simulink model "PassVeh14DOF"  (R2026b)
settings: Solver=ode23tb  StopTime=inf  FixedStep=.001  RelTol=1e-1  EnableMultiTasking=on
model workspace (MAT data in the model file):
  AlgnTrqCambCompl = [0 0 0 0]
  AlgnTrqSteerCompl = [0 0 0 0]
  AxlIxx = 62.3745166667
  AxlM = 160
  BumpCamber = [0 0 0 0]
  BumpCaster = [0 0 0 0]
  BumpSteer = [0 0 0 0]
  CambVsSteerAng = [0 0 0 0]
  CastVsSteerAng = [0 0 0 0]
  Cps = 2
  Cz = 5565.2246438
  CzWhlAxl = 11490.971257
  DCT_Param : object (value not decoded)
  Downshift_Speeds = [9.5625 12.9375 16.3125 19.6875 23.0625 26.4375 29.8125 33.1875 36.5625 39.9375 43.3125 46.6875 ... (28 elements, 4x7)]
  F0z = [2886 2907]
  F0zWhlAxl = 2907
  Hmax = 0.25
  Kz = 52451.0065793
  KzWhlAxl = 138031.612078
  LatCambCompl = [0 0 0 0]
  LatSteerCompl = [0 0 0 0]
  LatWhlCtrComplLat = [0 0 0 0]
  LatWhlCtrComplLng = [0  0  0  0; 0  0  0  0]
  LatWhlCtrDisp = [0 0 0 0]
  LngCambCompl = [0  0  0  0; 0  0  0  0]
  LngCastCompl = [0  0  0  0; 0  0  0  0]
  LngSteerCompl = [0  0  0  0; 0  0  0  0]
  LngWhlCtrCompl = [0  0  0  0; 0  0  0  0]
  LngWhlCtrDisp = [0 0 0 0]
  MotRatios = [1 1]
  NCyl = 6
  NrmlWhlFrcOff = [2886 2886 2907 2907]
  NrmlWhlRates = [52.4510065793 52.4510065793 52.4510065793 52.4510065793]
  Pedal_Positions = [0.1 0.4 0.5 0.9]
  Pstd = 101325
  Rair = 287
  RollCamber : object (value not decoded)
  RollCaster : object (value not decoded)
  RollSteer : object (value not decoded)
  RollStiffArb = [0 0]
  RollStiffArbFrnt = 800
  RollStiffNoArb = [0 0]
  RollStiffNoArbFrnt = 0
  RollStiffNoTwstRear = 0
  ShckFrcVsCompRate = [5.5652246438 5.5652246438 5.5652246438 5.5652246438]
  StatCamber = [0 0 0 0]
  StatCaster = [0 0 0 0]
  StatLdWhlR = [0.3 0.3 0.3 0.3]
  StatToe = [0 0 0 0]
  Trans : object (value not decoded)
  Tstd = 293.15
  Upshift_Speeds = [12.9375 16.3125 19.6875 33 26.4375 29.8125 33.1875 52.5 39.9375 43.3125 46.6875 77.25 ... (28 elements, 4x7)]
  VEH : object (value not decoded)
  Vd = 0.00346
  VrtLdTrnsfr = [0 0 0 0]
  WH : Mass (value not decoded)
  dt3D = 0.05
  f_air = [0 0 0 0 0 0 0 0 0 0 0 0 ... (256 elements, 16x16)]
  f_co = [0 0 0 0 0 0 0 0 0 0 0 0 ... (256 elements, 16x16)]
  f_co2 = [0 0 0 0 0 0 0 0 0 0 0 0 ... (256 elements, 16x16)]
  f_eff = [352.135682859 352.135682859 320.724378192 303.655312657 295.930136708 291.240087194 291.240271258 291.240312459 291.240275452 291.240198499 291.240100781 291.240018769 ... (256 elements, 16x16)]
  f_fuel = [0 0 0 0 0 0 0 0 0 0 0 0 ... (256 elements, 16x16)]
  f_hc = [0 0 0 0 0 0 0 0 0 0 0 0 ... (256 elements, 16x16)]
  f_nox = [0 0 0 0 0 0 0 0 0 0 0 0 ... (256 elements, 16x16)]
  f_pm = [0 0 0 0 0 0 0 0 0 0 0 0 ... (256 elements, 16x16)]
  f_susp_axl_bp = [1 2]
  f_susp_dz_bp = [-0.325022776267 -0.315022776267 -0.305022776267 -0.205022776267 -0.105022776267 -0.00502277626717 0.0949772237328 0.194977223733 0.204977223733 0.214977223733]
  f_susp_dzdot_bp = [-3 -0.3 -0.2 -0.1 0 0.1 0.2 0.3 3]
  f_susp_fmz = [-144070.391448 -93629.24037 -75929.1118915 -20630.5828179 -15385.48216 -10140.3815021 -4895.28084414 349.819813785 -31916.3973792 18437.6709544 -83996.1993354 -33555.0482577 ... (43920 elements, 10x9x61x2x4)]
  f_susp_geom = [0 0 0 0 0 0 0 0 0 0 0 0 ... (3660 elements, 10x61x2x3)]
  f_susp_strgdelta_bp = [-0.523598775598 -0.506145483078 -0.488692190558 -0.471238898038 -0.453785605519 -0.436332312999 -0.418879020479 -0.401425727959 -0.383972435439 -0.366519142919 -0.349065850399 -0.331612557879 ... (61 elements, 1x61)]
  f_tbrake = [0 76.8593923996 105.140482948 131.533638111 157.926793274 176.658631717 176.65727296 176.656856686 176.656879077 176.657093756 176.657404516 176.65772406 ... (256 elements, 16x16)]
  f_tbrake_n_bpt = [0 649.519052838 912.419621844 1175.32019085 1438.22075986 1701.12132886 1964.02189787 2226.92246687 2489.82303588 2752.72360489 3015.62417389 3278.5247429 ... (16 elements, 1x16)]
  f_tbrake_t_bpt = [0 34.6410161514 61.0341713143 87.4273264773 113.82048164 140.213636803 166.606791966 192.999947129 219.393102292 245.786257455 272.179412618 298.572567781 ... (16 elements, 1x16)]
  f_texh = [766.752464599 766.752464599 786.17542386 801.679939032 884.591982581 910.574397722 910.571871054 910.570774534 910.570601632 910.570821151 910.571247242 910.571639815 ... (256 elements, 16x16)]
  f_twc_eff_co = [0.17 0.25 0.45 0.99 0.99 0.99 0.99]
  f_twc_eff_hc = [0.21 0.375 0.75 0.98 0.98 0.98 0.98]
  f_twc_eff_lam = [0.909090909 0.944055944 0.979020979 1 1.013986014 1.048951049 1.083916084]
  f_twc_eff_nox = [0.98 0.98 0.98 0.97 0.05 0.02 0]
  numWheel = 4
symbols that are objects in the model workspace (value not decoded): VEH
libraries: vehdynlibtire x12, vehdynlibsuspension x8, autolibutils x5, sharedtransform x5, shared6dof x2, vehdynlibeom x1, vehdynlibtirecommon x1, matrix_library x1
(part 3 of 9)

== system PassVeh14DOF/Wheels and Tires/VDBS ==
  WhlAng : Inport
  WhlCmb : Inport  Port=2  Unit=rad
  AxleTrq : Inport  Port=3
  BrkPrs : Inport  Port=4
  Fz : Inport  Port=5  Unit=N
  r : Inport  Port=6
  VehVel : Inport  Port=7
  Ground Level : Inport  Port=8
  DCM : Inport  Port=9
  Friction : Inport  Port=10  Unit=1  PortDimensions=4
  Veh : Inport  Port=11
  Pressure : vehdynlibtirecommon/Constant  const=220000  numWheels=4
  Scale Factors : vehdynlibtire/Scale Factors  numWhls=4  LFZO=1  input_LFZO=off  LMUX=1  input_LMUX=on  LMUY=1  input_LMUY=on  LMUV=0  input_LMUV=off  LKX=1  input_LKX=off  LKY=1  input_LKY=off  LCX=1  input_LCX=off  LCY=1  input_LCY=off  LEX=1  input_LEX=off  LEY=1  input_LEY=off  LHX=1  input_LHX=off  LHY=1  input_LHY=off  LVX=1  input_LVX=off  LVY=1  input_LVY=off  LKYC=1  input_LKYC=off  LKZC=1  input_LKZC=off  LTR=1  input_LTR=off  LRES=1  input_LRES=off  LXAL=1  input_LXAL=off  LYKA=1  input_LYKA=off  LVYKA=1  input_LVYKA=off  LS=1  input_LS=off  LCZ=1  input_LCZ=off  LMX=1  input_LMX=off  LVMX=1  input_LVMX=off  LMY=1  input_LMY=off  LMP=1  input_LMP=off
  Terminator : Terminator
  Tire2Veh : Subsystem
  Tires : Subsystem  Variant=on  VariantControlMode=label  VariantControl=Variant1  LabelModeActiveChoice=2
  Veh2Tire : Subsystem
  Wheels : Outport  VectorParamsAs1DForOutWhenUnconnected=off
  Wheels2Susp : Outport  Port=2  VectorParamsAs1DForOutWhenUnconnected=off
  FrntAxlF : Outport  Port=3  Unit=N  VectorParamsAs1DForOutWhenUnconnected=off
  RearAxlF : Outport  Port=4  Unit=N  VectorParamsAs1DForOutWhenUnconnected=off
  Omega : Outport  Port=5  VectorParamsAs1DForOutWhenUnconnected=off
  Mz : Outport  Port=6  Unit=N*m  VectorParamsAs1DForOutWhenUnconnected=off
  SuspWhlPz : Outport  Port=7  VectorParamsAs1DForOutWhenUnconnected=off
  SuspWhlVz : Outport  Port=8  VectorParamsAs1DForOutWhenUnconnected=off
  wires:
  Ground Level/1 -> Tires/9("Gnd ")
  Pressure/1 -> Tires/7("Press ")
  Scale Factors/1 -> Tires/8("lambda ")
  Fz/1 -> Tire2Veh/3(Fz), Tires/10("FzSusp ")
  AxleTrq/1 -> Veh2Tire/2(Axle)
  BrkPrs/1 -> Veh2Tire/3(Brake)
  VehVel/1 -> Veh2Tire/4(VehVel)
  Veh2Tire/1(T) -> Tires/1("DriveTorque ")
  Veh2Tire/2(P) -> Tires/2("Brake Pressure ")
  Veh2Tire/4(xdotAxle) -> Tires/4("Vx ")
  Veh2Tire/5(ydotAxle) -> Tires/5("Vy ")
  Veh2Tire/3(psidot) -> Tires/3("r ")
  WhlAng/1 -> Tire2Veh/6(WhlAng), Veh2Tire/5(WhlAng)
  Tire2Veh/3(Omega) -> Omega/1
  Tire2Veh/4(FrntAxlF) -> FrntAxlF/1
  Tire2Veh/5(RearAxlF) -> RearAxlF/1
  Tire2Veh/6(<Mz>) -> Mz/1
  Friction/1 -> Scale Factors/2, Scale Factors/1
  r/1 -> Veh2Tire/1(r)
  Veh2Tire/6(zdotAxle) -> Terminator/1
  Tire2Veh/7(SuspWhlPz) -> SuspWhlPz/1
  Tire2Veh/8(SuspWhlVz) -> SuspWhlVz/1
  Veh/1 -> Tire2Veh/1(Veh)
  Tire2Veh/2(Wheels2Susp) -> Wheels2Susp/1
  Tires/1(" Wheels") -> Tire2Veh/2(Wheels)  "TireFrame"
  Tire2Veh/1(Wheel) -> Wheels/1
  WhlCmb/1 -> Veh2Tire/6(WhlCmb), Tire2Veh/5(WhlCmb)  "WhlCamberIn"
  Veh2Tire/7(Camber) -> Tires/6("Camber ")
  DCM/1 -> Veh2Tire/7(DCM), Tire2Veh/4(DCM)

== system PassVeh14DOF/Suspension/Double Wishbone Suspension/Steer Rate Adapter ==
  Veh : Inport
  Add : Sum
  Bus Selector3 : BusSelector  OutputSignals=BdyFrm.Cg.AngVel.r
  Constant : Constant  Value=zeros(1,4)
  Matrix Concatenate : Concatenate  NumInputs=3  Mode=Multidimensional array
  Matrix Concatenate1 : Concatenate  NumInputs=3  Mode=Multidimensional array
  Reshape2 : Reshape  OutputDimensionality=Row vector (2-D)
  Reshape3 : Reshape  OutputDimensionality=Row vector (2-D)
  Reshape4 : Reshape  OutputDimensionality=Row vector (2-D)
  Selector3 : Selector  InputPortWidth=1  IndexOptions=Index vector (dialog)  Indices=[1 1 1 1]  OutputSizes=1
  SteerRates : Constant  Value=zeros(1,4)
  AngVel : Outport  VectorParamsAs1DForOutWhenUnconnected=off
  wires:
  Reshape2/1 -> Matrix Concatenate1/1, Matrix Concatenate1/3, Matrix Concatenate1/2
  Constant/1 -> Reshape3/1
  Selector3/1 -> Reshape4/1
  Bus Selector3/1 -> Selector3/1  "<r>"
  Matrix Concatenate/1 -> Add/2
  SteerRates/1 -> Reshape2/1
  Reshape4/1 -> Matrix Concatenate/3
  Reshape3/1 -> Matrix Concatenate/2, Matrix Concatenate/1
  Matrix Concatenate1/1 -> Add/1
  Veh/1 -> Bus Selector3/1
  Add/1 -> AngVel/1  "AngVel"

== system PassVeh14DOF/Suspension/Double Wishbone Suspension/Steering Adapter ==
  Steer : Inport
  Reshape1 : Reshape  OutputDimensionality=Row vector (2-D)
  Selector : Selector  IndexOptions=Index vector (dialog)  Indices=[1 2]  OutputSizes=1
  StrgAng : Outport  VectorParamsAs1DForOutWhenUnconnected=off
  wires:
  Reshape1/1 -> StrgAng/1
  Steer/1 -> Selector/1
  Selector/1 -> Reshape1/1

== system PassVeh14DOF/Suspension/Double Wishbone Suspension/Vehicle Adapter ==
  Veh : Inport
  Bus Creator3 : BusCreator  Inputs=2
  Bus Selector1 : BusSelector  OutputSignals=InertFrm.FrntAxl.Lft.Disp.X,InertFrm.FrntAxl.Lft.Disp.Y,InertFrm.FrntAxl.Lft.Disp.Z,InertFrm.FrntAxl.Rght.Disp.X,InertFrm.FrntAxl.Rght.Disp.Y,InertFrm.FrntAxl.Rght.Disp.Z,InertFrm.RearAxl.Lft.Disp.X,InertFrm.RearAxl.Lft.Disp.Y,InertFrm.RearAxl.Lft.Disp.Z,InertFrm.RearAxl.Rght.Disp.X,InertFrm.RearAxl.Rght.Disp.Y,InertFrm.RearAxl.Rght.Disp.Z
  Bus Selector2 : BusSelector  OutputSignals=BdyFrm.FrntAxl.Lft.Vel.xdot,BdyFrm.FrntAxl.Lft.Vel.ydot,BdyFrm.FrntAxl.Lft.Vel.zdot,BdyFrm.FrntAxl.Rght.Vel.xdot,BdyFrm.FrntAxl.Rght.Vel.ydot,BdyFrm.FrntAxl.Rght.Vel.zdot,BdyFrm.RearAxl.Lft.Vel.xdot,BdyFrm.RearAxl.Lft.Vel.ydot,BdyFrm.RearAxl.Lft.Vel.zdot,BdyFrm.RearAxl.Rght.Vel.xdot,BdyFrm.RearAxl.Rght.Vel.ydot,BdyFrm.RearAxl.Rght.Vel.zdot
  Bus Selector3 : BusSelector  OutputSignals=InertFrm.FrntAxl.Lft.Vel.Xdot,InertFrm.FrntAxl.Lft.Vel.Ydot,InertFrm.FrntAxl.Lft.Vel.Zdot,InertFrm.FrntAxl.Rght.Vel.Xdot,InertFrm.FrntAxl.Rght.Vel.Ydot,InertFrm.FrntAxl.Rght.Vel.Zdot,InertFrm.RearAxl.Lft.Vel.Xdot,InertFrm.RearAxl.Lft.Vel.Ydot,InertFrm.RearAxl.Lft.Vel.Zdot,InertFrm.RearAxl.Rght.Vel.Xdot,InertFrm.RearAxl.Rght.Vel.Ydot,InertFrm.RearAxl.Rght.Vel.Zdot
  Inertial Frame CG to Axle Offset : Constant  Value=[zeros(2,4);VEH.HeightCG*ones(1,4)]
  Mux1 : Mux  Inputs=12
  Mux2 : Mux  Inputs=12
  Mux3 : Mux  Inputs=12
  Reshape : Reshape  OutputDimensionality=Customize  OutputDimensions=[3,4]
  Reshape1 : Reshape  OutputDimensionality=Customize  OutputDimensions=[3,4]
  Reshape2 : Reshape  OutputDimensionality=Customize  OutputDimensions=[3,4]
  Sum : Sum  Inputs=|+-
  VehSusp : Outport  VectorParamsAs1DForOutWhenUnconnected=off
  VehVbody : Outport  Port=2  VectorParamsAs1DForOutWhenUnconnected=off
  wires:
  Veh/1 -> Bus Selector3/1, Bus Selector2/1, Bus Selector1/1
  Reshape2/1 -> VehVbody/1  "V"
  Bus Creator3/1 -> VehSusp/1  "Veh"
  Reshape/1 -> Sum/1
  Bus Selector1/1 -> Mux2/1  "<X>"
  Bus Selector1/2 -> Mux2/2  "<Y>"
  Bus Selector1/3 -> Mux2/3  "<Z>"
  Bus Selector1/4 -> Mux2/4  "<X>"
  Bus Selector1/5 -> Mux2/5  "<Y>"
  Bus Selector1/6 -> Mux2/6  "<Z>"
  Bus Selector1/7 -> Mux2/7  "<X>"
  Bus Selector1/8 -> Mux2/8  "<Y>"
  Bus Selector1/9 -> Mux2/9  "<Z>"
  Bus Selector1/10 -> Mux2/10  "<X>"
  Bus Selector1/11 -> Mux2/11  "<Y>"
  Bus Selector1/12 -> Mux2/12  "<Z>"
  Bus Selector2/1 -> Mux1/1  "<xdot>"
  Bus Selector2/2 -> Mux1/2  "<ydot>"
  Bus Selector2/3 -> Mux1/3  "<zdot>"
  Bus Selector2/4 -> Mux1/4  "<xdot>"
  Bus Selector2/5 -> Mux1/5  "<ydot>"
  Bus Selector2/6 -> Mux1/6  "<zdot>"
  Bus Selector2/7 -> Mux1/7  "<xdot>"
  Bus Selector2/8 -> Mux1/8  "<ydot>"
  Bus Selector2/9 -> Mux1/9  "<zdot>"
  Bus Selector2/10 -> Mux1/10  "<xdot>"
  Bus Selector2/11 -> Mux1/11  "<ydot>"
  Bus Selector2/12 -> Mux1/12  "<zdot>"
  Mux1/1 -> Reshape2/1
  Mux2/1 -> Reshape/1
  Inertial Frame CG to Axle Offset/1 -> Sum/2
  Sum/1 -> Bus Creator3/1  "P"
  Mux3/1 -> Reshape1/1
  Bus Selector3/12 -> Mux3/12  "<Zdot>"
  Bus Selector3/11 -> Mux3/11  "<Ydot>"
  Bus Selector3/10 -> Mux3/10  "<Xdot>"
  Bus Selector3/9 -> Mux3/9  "<Zdot>"
  Bus Selector3/8 -> Mux3/8  "<Ydot>"
  Bus Selector3/7 -> Mux3/7  "<Xdot>"
  Bus Selector3/6 -> Mux3/6  "<Zdot>"
  Bus Selector3/5 -> Mux3/5  "<Ydot>"
  Bus Selector3/4 -> Mux3/4  "<Xdot>"
  Bus Selector3/3 -> Mux3/3  "<Zdot>"
  Bus Selector3/2 -> Mux3/2  "<Ydot>"
  Bus Selector3/1 -> Mux3/1  "<Xdot>"
  Reshape1/1 -> Bus Creator3/2  "V"

== system PassVeh14DOF/Suspension/Double Wishbone Suspension/Wheel  Adapter ==
  Wheels : Inport
  Bus Selector : BusSelector  OutputSignals=SuspFrame.Fx,SuspFrame.Fy
  Bus Selector1 : BusSelector  OutputSignals=SuspFrame.RL
  Bus Selector2 : BusSelector  OutputSignals=SuspFrame.Mx,SuspFrame.My,SuspFrame.Mz
  Bus Selector3 : BusSelector  OutputSignals=SuspFrame.z,SuspFrame.zdot
  Matrix Concatenate : Concatenate  NumInputs=3  Mode=Multidimensional array
  Reshape{,1..7} (8 alike) : Reshape  OutputDimensionality=Row vector (2-D)
  WhlFx : Outport  VectorParamsAs1DForOutWhenUnconnected=off
  WhlFy : Outport  Port=2  VectorParamsAs1DForOutWhenUnconnected=off
  z : Outport  Port=3  VectorParamsAs1DForOutWhenUnconnected=off
  zdot : Outport  Port=4  VectorParamsAs1DForOutWhenUnconnected=off
  M : Outport  Port=5  VectorParamsAs1DForOutWhenUnconnected=off
  RL : Outport  Port=6  VectorParamsAs1DForOutWhenUnconnected=off
  wires:
  Reshape7/1 -> WhlFy/1
  Reshape6/1 -> WhlFx/1
  Bus Selector/1 -> Reshape6/1  "<Fx>"
  Bus Selector/2 -> Reshape7/1  "<Fy>"
  Bus Selector3/1 -> Reshape/1  "<z>"
  Wheels/1 -> Bus Selector1/1, Bus Selector2/1, Bus Selector3/1, Bus Selector/1
  Bus Selector3/2 -> Reshape2/1  "<zdot>"
  Reshape2/1 -> zdot/1  "zdot"
  Bus Selector1/1 -> Reshape1/1  "<RL>"
  Reshape1/1 -> RL/1  "RL"
  Bus Selector2/1 -> Reshape3/1  "<Mx>"
  Bus Selector2/2 -> Reshape4/1  "<My>"
  Bus Selector2/3 -> Reshape5/1  "<Mz>"
  Reshape3/1 -> Matrix Concatenate/1
  Reshape4/1 -> Matrix Concatenate/2
  Reshape5/1 -> Matrix Concatenate/3
  Matrix Concatenate/1 -> M/1  "M"
  Reshape/1 -> z/1  "z"

== system PassVeh14DOF/Suspension/Independent Mapped Front Suspension Mapped Solid Axle Rear Suspension/Steer Rate Adapter ==
  Veh : Inport
  Add : Sum
  Bus Selector3 : BusSelector  OutputSignals=BdyFrm.Cg.AngVel.r
  Constant : Constant  Value=zeros(1,4)
  Matrix Concatenate : Concatenate  NumInputs=3  Mode=Multidimensional array
  Matrix Concatenate1 : Concatenate  NumInputs=3  Mode=Multidimensional array
  Reshape2 : Reshape  OutputDimensionality=Row vector (2-D)
  Reshape3 : Reshape  OutputDimensionality=Row vector (2-D)
  Reshape4 : Reshape  OutputDimensionality=Row vector (2-D)
  Selector3 : Selector  InputPortWidth=1  IndexOptions=Index vector (dialog)  Indices=[1 1 1 1]  OutputSizes=1
  SteerRates : Constant  Value=zeros(1,4)
  AngVel : Outport  VectorParamsAs1DForOutWhenUnconnected=off
  wires:
  Reshape2/1 -> Matrix Concatenate1/1, Matrix Concatenate1/3, Matrix Concatenate1/2
  Constant/1 -> Reshape3/1
  Selector3/1 -> Reshape4/1
  Bus Selector3/1 -> Selector3/1  "<r>"
  Matrix Concatenate/1 -> Add/2
  SteerRates/1 -> Reshape2/1
  Reshape4/1 -> Matrix Concatenate/3
  Reshape3/1 -> Matrix Concatenate/2, Matrix Concatenate/1
  Matrix Concatenate1/1 -> Add/1
  Veh/1 -> Bus Selector3/1
  Add/1 -> AngVel/1  "AngVel"

== system PassVeh14DOF/Suspension/Independent Mapped Front Suspension Mapped Solid Axle Rear Suspension/Steering Adapter ==
  Steer : Inport
  Reshape1 : Reshape  OutputDimensionality=Row vector (2-D)
  Selector : Selector  IndexOptions=Index vector (dialog)  Indices=[1 2]  OutputSizes=1
  StrgAng : Outport  VectorParamsAs1DForOutWhenUnconnected=off
  wires:
  Reshape1/1 -> StrgAng/1
  Steer/1 -> Selector/1
  Selector/1 -> Reshape1/1

== system PassVeh14DOF/Suspension/Independent Mapped Front Suspension Mapped Solid Axle Rear Suspension/Vehicle Adapter ==
  Veh : Inport
  Bus Creator3 : BusCreator  Inputs=2
  Bus Selector1 : BusSelector  OutputSignals=InertFrm.FrntAxl.Lft.Disp.X,InertFrm.FrntAxl.Lft.Disp.Y,InertFrm.FrntAxl.Lft.Disp.Z,InertFrm.FrntAxl.Rght.Disp.X,InertFrm.FrntAxl.Rght.Disp.Y,InertFrm.FrntAxl.Rght.Disp.Z,InertFrm.RearAxl.Lft.Disp.X,InertFrm.RearAxl.Lft.Disp.Y,InertFrm.RearAxl.Lft.Disp.Z,InertFrm.RearAxl.Rght.Disp.X,InertFrm.RearAxl.Rght.Disp.Y,InertFrm.RearAxl.Rght.Disp.Z
  Bus Selector2 : BusSelector  OutputSignals=BdyFrm.FrntAxl.Lft.Vel.xdot,BdyFrm.FrntAxl.Lft.Vel.ydot,BdyFrm.FrntAxl.Lft.Vel.zdot,BdyFrm.FrntAxl.Rght.Vel.xdot,BdyFrm.FrntAxl.Rght.Vel.ydot,BdyFrm.FrntAxl.Rght.Vel.zdot,BdyFrm.RearAxl.Lft.Vel.xdot,BdyFrm.RearAxl.Lft.Vel.ydot,BdyFrm.RearAxl.Lft.Vel.zdot,BdyFrm.RearAxl.Rght.Vel.xdot,BdyFrm.RearAxl.Rght.Vel.ydot,BdyFrm.RearAxl.Rght.Vel.zdot
  Bus Selector3 : BusSelector  OutputSignals=InertFrm.FrntAxl.Lft.Vel.Xdot,InertFrm.FrntAxl.Lft.Vel.Ydot,InertFrm.FrntAxl.Lft.Vel.Zdot,InertFrm.FrntAxl.Rght.Vel.Xdot,InertFrm.FrntAxl.Rght.Vel.Ydot,InertFrm.FrntAxl.Rght.Vel.Zdot,InertFrm.RearAxl.Lft.Vel.Xdot,InertFrm.RearAxl.Lft.Vel.Ydot,InertFrm.RearAxl.Lft.Vel.Zdot,InertFrm.RearAxl.Rght.Vel.Xdot,InertFrm.RearAxl.Rght.Vel.Ydot,InertFrm.RearAxl.Rght.Vel.Zdot
  Inertial Frame CG to Axle Offset : Constant  Value=[zeros(2,4);VEH.HeightCG*ones(1,4)]
  Mux1 : Mux  Inputs=12
  Mux2 : Mux  Inputs=12
  Mux3 : Mux  Inputs=12
  Reshape : Reshape  OutputDimensionality=Customize  OutputDimensions=[3,4]
  Reshape1 : Reshape  OutputDimensionality=Customize  OutputDimensions=[3,4]
  Reshape2 : Reshape  OutputDimensionality=Customize  OutputDimensions=[3,4]
  Sum : Sum  Inputs=|+-
  VehSusp : Outport  VectorParamsAs1DForOutWhenUnconnected=off
  VehVbody : Outport  Port=2  VectorParamsAs1DForOutWhenUnconnected=off
  wires:
  Veh/1 -> Bus Selector3/1, Bus Selector2/1, Bus Selector1/1
  Reshape2/1 -> VehVbody/1  "V"
  Bus Creator3/1 -> VehSusp/1  "Veh"
  Reshape/1 -> Sum/1
  Bus Selector1/1 -> Mux2/1  "<X>"
  Bus Selector1/2 -> Mux2/2  "<Y>"
  Bus Selector1/3 -> Mux2/3  "<Z>"
  Bus Selector1/4 -> Mux2/4  "<X>"
  Bus Selector1/5 -> Mux2/5  "<Y>"
  Bus Selector1/6 -> Mux2/6  "<Z>"
  Bus Selector1/7 -> Mux2/7  "<X>"
  Bus Selector1/8 -> Mux2/8  "<Y>"
  Bus Selector1/9 -> Mux2/9  "<Z>"
  Bus Selector1/10 -> Mux2/10  "<X>"
  Bus Selector1/11 -> Mux2/11  "<Y>"
  Bus Selector1/12 -> Mux2/12  "<Z>"
  Bus Selector2/1 -> Mux1/1  "<xdot>"
  Bus Selector2/2 -> Mux1/2  "<ydot>"
  Bus Selector2/3 -> Mux1/3  "<zdot>"
  Bus Selector2/4 -> Mux1/4  "<xdot>"
  Bus Selector2/5 -> Mux1/5  "<ydot>"
  Bus Selector2/6 -> Mux1/6  "<zdot>"
  Bus Selector2/7 -> Mux1/7  "<xdot>"
  Bus Selector2/8 -> Mux1/8  "<ydot>"
  Bus Selector2/9 -> Mux1/9  "<zdot>"
  Bus Selector2/10 -> Mux1/10  "<xdot>"
  Bus Selector2/11 -> Mux1/11  "<ydot>"
  Bus Selector2/12 -> Mux1/12  "<zdot>"
  Mux1/1 -> Reshape2/1
  Mux2/1 -> Reshape/1
  Inertial Frame CG to Axle Offset/1 -> Sum/2
  Sum/1 -> Bus Creator3/1  "P"
  Mux3/1 -> Reshape1/1
  Bus Selector3/12 -> Mux3/12  "<Zdot>"
  Bus Selector3/11 -> Mux3/11  "<Ydot>"
  Bus Selector3/10 -> Mux3/10  "<Xdot>"
  Bus Selector3/9 -> Mux3/9  "<Zdot>"
  Bus Selector3/8 -> Mux3/8  "<Ydot>"
  Bus Selector3/7 -> Mux3/7  "<Xdot>"
  Bus Selector3/6 -> Mux3/6  "<Zdot>"
  Bus Selector3/5 -> Mux3/5  "<Ydot>"
  Bus Selector3/4 -> Mux3/4  "<Xdot>"
  Bus Selector3/3 -> Mux3/3  "<Zdot>"
  Bus Selector3/2 -> Mux3/2  "<Ydot>"
  Bus Selector3/1 -> Mux3/1  "<Xdot>"
  Reshape1/1 -> Bus Creator3/2  "V"

== system PassVeh14DOF/Suspension/Independent Mapped Front Suspension Mapped Solid Axle Rear Suspension/Wheel  Adapter ==
  Wheels : Inport
  Bus Selector : BusSelector  OutputSignals=SuspFrame.Fx,SuspFrame.Fy
  Bus Selector1 : BusSelector  OutputSignals=SuspFrame.RL
  Bus Selector2 : BusSelector  OutputSignals=SuspFrame.Mx,SuspFrame.My,SuspFrame.Mz
  Bus Selector3 : BusSelector  OutputSignals=SuspFrame.z,SuspFrame.zdot
  Matrix Concatenate : Concatenate  NumInputs=3  Mode=Multidimensional array
  Reshape{,1..7} (8 alike) : Reshape  OutputDimensionality=Row vector (2-D)
  WhlFx : Outport  VectorParamsAs1DForOutWhenUnconnected=off
  WhlFy : Outport  Port=2  VectorParamsAs1DForOutWhenUnconnected=off
  z : Outport  Port=3  VectorParamsAs1DForOutWhenUnconnected=off
  zdot : Outport  Port=4  VectorParamsAs1DForOutWhenUnconnected=off
  M : Outport  Port=5  VectorParamsAs1DForOutWhenUnconnected=off
  RL : Outport  Port=6  VectorParamsAs1DForOutWhenUnconnected=off
  wires:
  Reshape7/1 -> WhlFy/1
  Reshape6/1 -> WhlFx/1
  Bus Selector/1 -> Reshape6/1  "<Fx>"
  Bus Selector/2 -> Reshape7/1  "<Fy>"
  Bus Selector3/1 -> Reshape/1  "<z>"
  Wheels/1 -> Bus Selector1/1, Bus Selector2/1, Bus Selector3/1, Bus Selector/1
  Bus Selector3/2 -> Reshape2/1  "<zdot>"
  Reshape2/1 -> zdot/1  "zdot"
  Bus Selector1/1 -> Reshape1/1  "<RL>"
  Reshape1/1 -> RL/1  "RL"
  Bus Selector2/1 -> Reshape3/1  "<Mx>"
  Bus Selector2/2 -> Reshape4/1  "<My>"
  Bus Selector2/3 -> Reshape5/1  "<Mz>"
  Reshape3/1 -> Matrix Concatenate/1
  Reshape4/1 -> Matrix Concatenate/2
  Reshape5/1 -> Matrix Concatenate/3
  Matrix Concatenate/1 -> M/1  "M"
  Reshape/1 -> z/1  "z"

== system PassVeh14DOF/Suspension/Kinematics and Compliance Independent Suspension/Calculate dynamic track width from lateral wheel center displacement change ==
  dWhlY : Inport
  dWhlZ : Inport  Port=2
  Front Track Calculation : Subsystem
  Gain : Gain  Gain=-1
  Rear Track Calculation : Subsystem
  Sign : Signum  ZeroCross=off
  Vector Concatenate : Concatenate
  w : Outport
  wires:
  dWhlZ/1 -> Gain/1
  dWhlY/1 -> Rear Track Calculation/1(dWhlY), Front Track Calculation/1(dWhlY)
  Vector Concatenate/1 -> w/1
  Front Track Calculation/1(w_front) -> Vector Concatenate/1
  Rear Track Calculation/1(w_rear) -> Vector Concatenate/2
  Sign/1 -> Rear Track Calculation/2(sign), Front Track Calculation/2(sign)
  Gain/1 -> Sign/1

== system PassVeh14DOF/Suspension/Kinematics and Compliance Independent Suspension/Steer Rate Adapter ==
  Veh : Inport
  Add : Sum
  Bus Selector3 : BusSelector  OutputSignals=BdyFrm.Cg.AngVel.r
  Constant : Constant  Value=zeros(1,4)
  Matrix Concatenate : Concatenate  NumInputs=3  Mode=Multidimensional array
  Matrix Concatenate1 : Concatenate  NumInputs=3  Mode=Multidimensional array
  Reshape2 : Reshape  OutputDimensionality=Row vector (2-D)
  Reshape3 : Reshape  OutputDimensionality=Row vector (2-D)
  Reshape4 : Reshape  OutputDimensionality=Row vector (2-D)
  Selector3 : Selector  InputPortWidth=1  IndexOptions=Index vector (dialog)  Indices=[1 1 1 1]  OutputSizes=1
  SteerRates : Constant  Value=zeros(1,4)
  AngVel : Outport  VectorParamsAs1DForOutWhenUnconnected=off
  wires:
  Reshape2/1 -> Matrix Concatenate1/1, Matrix Concatenate1/3, Matrix Concatenate1/2
  Constant/1 -> Reshape3/1
  Selector3/1 -> Reshape4/1
  Bus Selector3/1 -> Selector3/1  "<r>"
  Matrix Concatenate/1 -> Add/2
  SteerRates/1 -> Reshape2/1
  Reshape4/1 -> Matrix Concatenate/3
  Reshape3/1 -> Matrix Concatenate/2, Matrix Concatenate/1
  Matrix Concatenate1/1 -> Add/1
  Veh/1 -> Bus Selector3/1
  Add/1 -> AngVel/1  "AngVel"

== system PassVeh14DOF/Suspension/Kinematics and Compliance Independent Suspension/Steering Adapter ==
  Steer : Inport
  Reshape1 : Reshape  OutputDimensionality=Row vector (2-D)
  Selector : Selector  IndexOptions=Index vector (dialog)  Indices=[1 2]  OutputSizes=1
  StrgAng : Outport  VectorParamsAs1DForOutWhenUnconnected=off
  wires:
  Reshape1/1 -> StrgAng/1
  Steer/1 -> Selector/1
  Selector/1 -> Reshape1/1

== system PassVeh14DOF/Suspension/Kinematics and Compliance Independent Suspension/Vehicle Adapter ==
  Veh : Inport
  Bus Creator3 : BusCreator  Inputs=2
  Bus Selector1 : BusSelector  OutputSignals=InertFrm.FrntAxl.Lft.Disp.X,InertFrm.FrntAxl.Lft.Disp.Y,InertFrm.FrntAxl.Lft.Disp.Z,InertFrm.FrntAxl.Rght.Disp.X,InertFrm.FrntAxl.Rght.Disp.Y,InertFrm.FrntAxl.Rght.Disp.Z,InertFrm.RearAxl.Lft.Disp.X,InertFrm.RearAxl.Lft.Disp.Y,InertFrm.RearAxl.Lft.Disp.Z,InertFrm.RearAxl.Rght.Disp.X,InertFrm.RearAxl.Rght.Disp.Y,InertFrm.RearAxl.Rght.Disp.Z
  Bus Selector2 : BusSelector  OutputSignals=BdyFrm.FrntAxl.Lft.Vel.xdot,BdyFrm.FrntAxl.Lft.Vel.ydot,BdyFrm.FrntAxl.Lft.Vel.zdot,BdyFrm.FrntAxl.Rght.Vel.xdot,BdyFrm.FrntAxl.Rght.Vel.ydot,BdyFrm.FrntAxl.Rght.Vel.zdot,BdyFrm.RearAxl.Lft.Vel.xdot,BdyFrm.RearAxl.Lft.Vel.ydot,BdyFrm.RearAxl.Lft.Vel.zdot,BdyFrm.RearAxl.Rght.Vel.xdot,BdyFrm.RearAxl.Rght.Vel.ydot,BdyFrm.RearAxl.Rght.Vel.zdot
  Bus Selector3 : BusSelector  OutputSignals=InertFrm.FrntAxl.Lft.Vel.Xdot,InertFrm.FrntAxl.Lft.Vel.Ydot,InertFrm.FrntAxl.Lft.Vel.Zdot,InertFrm.FrntAxl.Rght.Vel.Xdot,InertFrm.FrntAxl.Rght.Vel.Ydot,InertFrm.FrntAxl.Rght.Vel.Zdot,InertFrm.RearAxl.Lft.Vel.Xdot,InertFrm.RearAxl.Lft.Vel.Ydot,InertFrm.RearAxl.Lft.Vel.Zdot,InertFrm.RearAxl.Rght.Vel.Xdot,InertFrm.RearAxl.Rght.Vel.Ydot,InertFrm.RearAxl.Rght.Vel.Zdot
  Inertial Frame CG to Axle Offset : Constant  Value=[zeros(2,4);VEH.HeightCG*ones(1,4)]
  Mux1 : Mux  Inputs=12
  Mux2 : Mux  Inputs=12
  Mux3 : Mux  Inputs=12
  Reshape : Reshape  OutputDimensionality=Customize  OutputDimensions=[3,4]
  Reshape1 : Reshape  OutputDimensionality=Customize  OutputDimensions=[3,4]
  Reshape2 : Reshape  OutputDimensionality=Customize  OutputDimensions=[3,4]
  Sum : Sum  Inputs=|+-
  VehSusp : Outport  VectorParamsAs1DForOutWhenUnconnected=off
  VehVbody : Outport  Port=2  VectorParamsAs1DForOutWhenUnconnected=off
  wires:
  Veh/1 -> Bus Selector3/1, Bus Selector2/1, Bus Selector1/1
  Reshape2/1 -> VehVbody/1  "V"
  Bus Creator3/1 -> VehSusp/1  "Veh"
  Reshape/1 -> Sum/1
  Bus Selector1/1 -> Mux2/1  "<X>"
  Bus Selector1/2 -> Mux2/2  "<Y>"
  Bus Selector1/3 -> Mux2/3  "<Z>"
  Bus Selector1/4 -> Mux2/4  "<X>"
  Bus Selector1/5 -> Mux2/5  "<Y>"
  Bus Selector1/6 -> Mux2/6  "<Z>"
  Bus Selector1/7 -> Mux2/7  "<X>"
  Bus Selector1/8 -> Mux2/8  "<Y>"
  Bus Selector1/9 -> Mux2/9  "<Z>"
  Bus Selector1/10 -> Mux2/10  "<X>"
  Bus Selector1/11 -> Mux2/11  "<Y>"
  Bus Selector1/12 -> Mux2/12  "<Z>"
  Bus Selector2/1 -> Mux1/1  "<xdot>"
  Bus Selector2/2 -> Mux1/2  "<ydot>"
  Bus Selector2/3 -> Mux1/3  "<zdot>"
  Bus Selector2/4 -> Mux1/4  "<xdot>"
  Bus Selector2/5 -> Mux1/5  "<ydot>"
  Bus Selector2/6 -> Mux1/6  "<zdot>"
  Bus Selector2/7 -> Mux1/7  "<xdot>"
  Bus Selector2/8 -> Mux1/8  "<ydot>"
  Bus Selector2/9 -> Mux1/9  "<zdot>"
  Bus Selector2/10 -> Mux1/10  "<xdot>"
  Bus Selector2/11 -> Mux1/11  "<ydot>"
  Bus Selector2/12 -> Mux1/12  "<zdot>"
  Mux1/1 -> Reshape2/1
  Mux2/1 -> Reshape/1
  Inertial Frame CG to Axle Offset/1 -> Sum/2
  Sum/1 -> Bus Creator3/1  "P"
  Mux3/1 -> Reshape1/1
  Bus Selector3/12 -> Mux3/12  "<Zdot>"
  Bus Selector3/11 -> Mux3/11  "<Ydot>"
  Bus Selector3/10 -> Mux3/10  "<Xdot>"
  Bus Selector3/9 -> Mux3/9  "<Zdot>"
  Bus Selector3/8 -> Mux3/8  "<Ydot>"
  Bus Selector3/7 -> Mux3/7  "<Xdot>"
  Bus Selector3/6 -> Mux3/6  "<Zdot>"
  Bus Selector3/5 -> Mux3/5  "<Ydot>"
  Bus Selector3/4 -> Mux3/4  "<Xdot>"
  Bus Selector3/3 -> Mux3/3  "<Zdot>"
  Bus Selector3/2 -> Mux3/2  "<Ydot>"
  Bus Selector3/1 -> Mux3/1  "<Xdot>"
  Reshape1/1 -> Bus Creator3/2  "V"

== system PassVeh14DOF/Suspension/Kinematics and Compliance Independent Suspension/Wheel  Adapter ==
  Wheels : Inport
  Bus Selector : BusSelector  OutputSignals=SuspFrame.Fx,SuspFrame.Fy
  Bus Selector1 : BusSelector  OutputSignals=SuspFrame.RL
  Bus Selector2 : BusSelector  OutputSignals=SuspFrame.Mx,SuspFrame.My,SuspFrame.Mz
  Bus Selector3 : BusSelector  OutputSignals=SuspFrame.z,SuspFrame.zdot
  Matrix Concatenate : Concatenate  NumInputs=3  Mode=Multidimensional array
  Reshape{,1..7} (8 alike) : Reshape  OutputDimensionality=Row vector (2-D)
  WhlFx : Outport  VectorParamsAs1DForOutWhenUnconnected=off
  WhlFy : Outport  Port=2  VectorParamsAs1DForOutWhenUnconnected=off
  z : Outport  Port=3  VectorParamsAs1DForOutWhenUnconnected=off
  zdot : Outport  Port=4  VectorParamsAs1DForOutWhenUnconnected=off
  M : Outport  Port=5  VectorParamsAs1DForOutWhenUnconnected=off
  RL : Outport  Port=6  VectorParamsAs1DForOutWhenUnconnected=off
  wires:
  Reshape7/1 -> WhlFy/1
  Reshape6/1 -> WhlFx/1
  Bus Selector/1 -> Reshape6/1  "<Fx>"
  Bus Selector/2 -> Reshape7/1  "<Fy>"
  Bus Selector3/1 -> Reshape/1  "<z>"
  Wheels/1 -> Bus Selector1/1, Bus Selector2/1, Bus Selector3/1, Bus Selector/1
  Bus Selector3/2 -> Reshape2/1  "<zdot>"
  Reshape2/1 -> zdot/1  "zdot"
  Bus Selector1/1 -> Reshape1/1  "<RL>"
  Reshape1/1 -> RL/1  "RL"
  Bus Selector2/1 -> Reshape3/1  "<Mx>"
  Bus Selector2/2 -> Reshape4/1  "<My>"
  Bus Selector2/3 -> Reshape5/1  "<Mz>"
  Reshape3/1 -> Matrix Concatenate/1
  Reshape4/1 -> Matrix Concatenate/2
  Reshape5/1 -> Matrix Concatenate/3
  Matrix Concatenate/1 -> M/1  "M"
  Reshape/1 -> z/1  "z"

== system PassVeh14DOF/Suspension/MacPherson Front Suspension Solid Axle Rear Suspension/Steer Rate Adapter ==
  Veh : Inport
  Add : Sum
  Bus Selector3 : BusSelector  OutputSignals=BdyFrm.Cg.AngVel.r
  Constant : Constant  Value=zeros(1,4)
  Matrix Concatenate : Concatenate  NumInputs=3  Mode=Multidimensional array
  Matrix Concatenate1 : Concatenate  NumInputs=3  Mode=Multidimensional array
  Reshape2 : Reshape  OutputDimensionality=Row vector (2-D)
  Reshape3 : Reshape  OutputDimensionality=Row vector (2-D)
  Reshape4 : Reshape  OutputDimensionality=Row vector (2-D)
  Selector3 : Selector  InputPortWidth=1  IndexOptions=Index vector (dialog)  Indices=[1 1 1 1]  OutputSizes=1
  SteerRates : Constant  Value=zeros(1,4)
  AngVel : Outport  VectorParamsAs1DForOutWhenUnconnected=off
  wires:
  Reshape2/1 -> Matrix Concatenate1/1, Matrix Concatenate1/3, Matrix Concatenate1/2
  Constant/1 -> Reshape3/1
  Selector3/1 -> Reshape4/1
  Bus Selector3/1 -> Selector3/1  "<r>"
  Matrix Concatenate/1 -> Add/2
  SteerRates/1 -> Reshape2/1
  Reshape4/1 -> Matrix Concatenate/3
  Reshape3/1 -> Matrix Concatenate/2, Matrix Concatenate/1
  Matrix Concatenate1/1 -> Add/1
  Veh/1 -> Bus Selector3/1
  Add/1 -> AngVel/1  "AngVel"

== system PassVeh14DOF/Suspension/MacPherson Front Suspension Solid Axle Rear Suspension/Steering Adapter ==
  Steer : Inport
  Reshape1 : Reshape  OutputDimensionality=Row vector (2-D)
  Selector : Selector  IndexOptions=Index vector (dialog)  Indices=[1 2]  OutputSizes=1
  StrgAng : Outport  VectorParamsAs1DForOutWhenUnconnected=off
  wires:
  Reshape1/1 -> StrgAng/1
  Steer/1 -> Selector/1
  Selector/1 -> Reshape1/1

== system PassVeh14DOF/Suspension/MacPherson Front Suspension Solid Axle Rear Suspension/Vehicle Adapter ==
  Veh : Inport
  Bus Creator3 : BusCreator  Inputs=2
  Bus Selector1 : BusSelector  OutputSignals=InertFrm.FrntAxl.Lft.Disp.X,InertFrm.FrntAxl.Lft.Disp.Y,InertFrm.FrntAxl.Lft.Disp.Z,InertFrm.FrntAxl.Rght.Disp.X,InertFrm.FrntAxl.Rght.Disp.Y,InertFrm.FrntAxl.Rght.Disp.Z,InertFrm.RearAxl.Lft.Disp.X,InertFrm.RearAxl.Lft.Disp.Y,InertFrm.RearAxl.Lft.Disp.Z,InertFrm.RearAxl.Rght.Disp.X,InertFrm.RearAxl.Rght.Disp.Y,InertFrm.RearAxl.Rght.Disp.Z
  Bus Selector2 : BusSelector  OutputSignals=BdyFrm.FrntAxl.Lft.Vel.xdot,BdyFrm.FrntAxl.Lft.Vel.ydot,BdyFrm.FrntAxl.Lft.Vel.zdot,BdyFrm.FrntAxl.Rght.Vel.xdot,BdyFrm.FrntAxl.Rght.Vel.ydot,BdyFrm.FrntAxl.Rght.Vel.zdot,BdyFrm.RearAxl.Lft.Vel.xdot,BdyFrm.RearAxl.Lft.Vel.ydot,BdyFrm.RearAxl.Lft.Vel.zdot,BdyFrm.RearAxl.Rght.Vel.xdot,BdyFrm.RearAxl.Rght.Vel.ydot,BdyFrm.RearAxl.Rght.Vel.zdot
  Bus Selector3 : BusSelector  OutputSignals=InertFrm.FrntAxl.Lft.Vel.Xdot,InertFrm.FrntAxl.Lft.Vel.Ydot,InertFrm.FrntAxl.Lft.Vel.Zdot,InertFrm.FrntAxl.Rght.Vel.Xdot,InertFrm.FrntAxl.Rght.Vel.Ydot,InertFrm.FrntAxl.Rght.Vel.Zdot,InertFrm.RearAxl.Lft.Vel.Xdot,InertFrm.RearAxl.Lft.Vel.Ydot,InertFrm.RearAxl.Lft.Vel.Zdot,InertFrm.RearAxl.Rght.Vel.Xdot,InertFrm.RearAxl.Rght.Vel.Ydot,InertFrm.RearAxl.Rght.Vel.Zdot
  Inertial Frame CG to Axle Offset : Constant  Value=[zeros(2,4);VEH.HeightCG*ones(1,4)]
  Mux1 : Mux  Inputs=12
  Mux2 : Mux  Inputs=12
  Mux3 : Mux  Inputs=12
  Reshape : Reshape  OutputDimensionality=Customize  OutputDimensions=[3,4]
  Reshape1 : Reshape  OutputDimensionality=Customize  OutputDimensions=[3,4]
  Reshape2 : Reshape  OutputDimensionality=Customize  OutputDimensions=[3,4]
  Sum : Sum  Inputs=|+-
  VehSusp : Outport  VectorParamsAs1DForOutWhenUnconnected=off
  VehVbody : Outport  Port=2  VectorParamsAs1DForOutWhenUnconnected=off
  wires:
  Veh/1 -> Bus Selector3/1, Bus Selector2/1, Bus Selector1/1
  Reshape2/1 -> VehVbody/1  "V"
  Bus Creator3/1 -> VehSusp/1  "Veh"
  Reshape/1 -> Sum/1
  Bus Selector1/1 -> Mux2/1  "<X>"
  Bus Selector1/2 -> Mux2/2  "<Y>"
  Bus Selector1/3 -> Mux2/3  "<Z>"
  Bus Selector1/4 -> Mux2/4  "<X>"
  Bus Selector1/5 -> Mux2/5  "<Y>"
  Bus Selector1/6 -> Mux2/6  "<Z>"
  Bus Selector1/7 -> Mux2/7  "<X>"
  Bus Selector1/8 -> Mux2/8  "<Y>"
  Bus Selector1/9 -> Mux2/9  "<Z>"
  Bus Selector1/10 -> Mux2/10  "<X>"
  Bus Selector1/11 -> Mux2/11  "<Y>"
  Bus Selector1/12 -> Mux2/12  "<Z>"
  Bus Selector2/1 -> Mux1/1  "<xdot>"
  Bus Selector2/2 -> Mux1/2  "<ydot>"
  Bus Selector2/3 -> Mux1/3  "<zdot>"
  Bus Selector2/4 -> Mux1/4  "<xdot>"
  Bus Selector2/5 -> Mux1/5  "<ydot>"
  Bus Selector2/6 -> Mux1/6  "<zdot>"
  Bus Selector2/7 -> Mux1/7  "<xdot>"
  Bus Selector2/8 -> Mux1/8  "<ydot>"
  Bus Selector2/9 -> Mux1/9  "<zdot>"
  Bus Selector2/10 -> Mux1/10  "<xdot>"
  Bus Selector2/11 -> Mux1/11  "<ydot>"
  Bus Selector2/12 -> Mux1/12  "<zdot>"
  Mux1/1 -> Reshape2/1
  Mux2/1 -> Reshape/1
  Inertial Frame CG to Axle Offset/1 -> Sum/2
  Sum/1 -> Bus Creator3/1  "P"
  Mux3/1 -> Reshape1/1
  Bus Selector3/12 -> Mux3/12  "<Zdot>"
  Bus Selector3/11 -> Mux3/11  "<Ydot>"
  Bus Selector3/10 -> Mux3/10  "<Xdot>"
  Bus Selector3/9 -> Mux3/9  "<Zdot>"
  Bus Selector3/8 -> Mux3/8  "<Ydot>"
  Bus Selector3/7 -> Mux3/7  "<Xdot>"
  Bus Selector3/6 -> Mux3/6  "<Zdot>"
  Bus Selector3/5 -> Mux3/5  "<Ydot>"
  Bus Selector3/4 -> Mux3/4  "<Xdot>"
  Bus Selector3/3 -> Mux3/3  "<Zdot>"
  Bus Selector3/2 -> Mux3/2  "<Ydot>"
  Bus Selector3/1 -> Mux3/1  "<Xdot>"
  Reshape1/1 -> Bus Creator3/2  "V"

== system PassVeh14DOF/Suspension/MacPherson Front Suspension Solid Axle Rear Suspension/Wheel  Adapter ==
  Wheels : Inport
  Bus Selector : BusSelector  OutputSignals=SuspFrame.Fx,SuspFrame.Fy
  Bus Selector1 : BusSelector  OutputSignals=SuspFrame.RL
  Bus Selector2 : BusSelector  OutputSignals=SuspFrame.Mx,SuspFrame.My,SuspFrame.Mz
  Bus Selector3 : BusSelector  OutputSignals=SuspFrame.z,SuspFrame.zdot
  Matrix Concatenate : Concatenate  NumInputs=3  Mode=Multidimensional array
  Reshape{,1..7} (8 alike) : Reshape  OutputDimensionality=Row vector (2-D)
  WhlFx : Outport  VectorParamsAs1DForOutWhenUnconnected=off
  WhlFy : Outport  Port=2  VectorParamsAs1DForOutWhenUnconnected=off
  z : Outport  Port=3  VectorParamsAs1DForOutWhenUnconnected=off
  zdot : Outport  Port=4  VectorParamsAs1DForOutWhenUnconnected=off
  M : Outport  Port=5  VectorParamsAs1DForOutWhenUnconnected=off
  RL : Outport  Port=6  VectorParamsAs1DForOutWhenUnconnected=off
  wires:
  Reshape7/1 -> WhlFy/1
  Reshape6/1 -> WhlFx/1
  Bus Selector/1 -> Reshape6/1  "<Fx>"
  Bus Selector/2 -> Reshape7/1  "<Fy>"
  Bus Selector3/1 -> Reshape/1  "<z>"
  Wheels/1 -> Bus Selector1/1, Bus Selector2/1, Bus Selector3/1, Bus Selector/1
  Bus Selector3/2 -> Reshape2/1  "<zdot>"
  Reshape2/1 -> zdot/1  "zdot"
  Bus Selector1/1 -> Reshape1/1  "<RL>"
  Reshape1/1 -> RL/1  "RL"
  Bus Selector2/1 -> Reshape3/1  "<Mx>"
  Bus Selector2/2 -> Reshape4/1  "<My>"
  Bus Selector2/3 -> Reshape5/1  "<Mz>"
  Reshape3/1 -> Matrix Concatenate/1
  Reshape4/1 -> Matrix Concatenate/2
  Reshape5/1 -> Matrix Concatenate/3
  Matrix Concatenate/1 -> M/1  "M"
  Reshape/1 -> z/1  "z"

== system PassVeh14DOF/Suspension/MacPherson Suspension/Steer Rate Adapter ==
  Veh : Inport
  Add : Sum
  Bus Selector3 : BusSelector  OutputSignals=BdyFrm.Cg.AngVel.r
  Constant : Constant  Value=zeros(1,4)
  Matrix Concatenate : Concatenate  NumInputs=3  Mode=Multidimensional array
  Matrix Concatenate1 : Concatenate  NumInputs=3  Mode=Multidimensional array
  Reshape2 : Reshape  OutputDimensionality=Row vector (2-D)
  Reshape3 : Reshape  OutputDimensionality=Row vector (2-D)
  Reshape4 : Reshape  OutputDimensionality=Row vector (2-D)
  Selector3 : Selector  InputPortWidth=1  IndexOptions=Index vector (dialog)  Indices=[1 1 1 1]  OutputSizes=1
  SteerRates : Constant  Value=zeros(1,4)
  AngVel : Outport  VectorParamsAs1DForOutWhenUnconnected=off
  wires:
  Reshape2/1 -> Matrix Concatenate1/1, Matrix Concatenate1/3, Matrix Concatenate1/2
  Constant/1 -> Reshape3/1
  Selector3/1 -> Reshape4/1
  Bus Selector3/1 -> Selector3/1  "<r>"
  Matrix Concatenate/1 -> Add/2
  SteerRates/1 -> Reshape2/1
  Reshape4/1 -> Matrix Concatenate/3
  Reshape3/1 -> Matrix Concatenate/2, Matrix Concatenate/1
  Matrix Concatenate1/1 -> Add/1
  Veh/1 -> Bus Selector3/1
  Add/1 -> AngVel/1  "AngVel"

== system PassVeh14DOF/Suspension/MacPherson Suspension/Steering Adapter ==
  Steer : Inport
  Reshape1 : Reshape  OutputDimensionality=Row vector (2-D)
  Selector : Selector  IndexOptions=Index vector (dialog)  Indices=[1 2]  OutputSizes=1
  StrgAng : Outport  VectorParamsAs1DForOutWhenUnconnected=off
  wires:
  Reshape1/1 -> StrgAng/1
  Steer/1 -> Selector/1
  Selector/1 -> Reshape1/1

== system PassVeh14DOF/Suspension/MacPherson Suspension/Vehicle Adapter ==
  Veh : Inport
  Bus Creator3 : BusCreator  Inputs=2
  Bus Selector1 : BusSelector  OutputSignals=InertFrm.FrntAxl.Lft.Disp.X,InertFrm.FrntAxl.Lft.Disp.Y,InertFrm.FrntAxl.Lft.Disp.Z,InertFrm.FrntAxl.Rght.Disp.X,InertFrm.FrntAxl.Rght.Disp.Y,InertFrm.FrntAxl.Rght.Disp.Z,InertFrm.RearAxl.Lft.Disp.X,InertFrm.RearAxl.Lft.Disp.Y,InertFrm.RearAxl.Lft.Disp.Z,InertFrm.RearAxl.Rght.Disp.X,InertFrm.RearAxl.Rght.Disp.Y,InertFrm.RearAxl.Rght.Disp.Z
  Bus Selector2 : BusSelector  OutputSignals=BdyFrm.FrntAxl.Lft.Vel.xdot,BdyFrm.FrntAxl.Lft.Vel.ydot,BdyFrm.FrntAxl.Lft.Vel.zdot,BdyFrm.FrntAxl.Rght.Vel.xdot,BdyFrm.FrntAxl.Rght.Vel.ydot,BdyFrm.FrntAxl.Rght.Vel.zdot,BdyFrm.RearAxl.Lft.Vel.xdot,BdyFrm.RearAxl.Lft.Vel.ydot,BdyFrm.RearAxl.Lft.Vel.zdot,BdyFrm.RearAxl.Rght.Vel.xdot,BdyFrm.RearAxl.Rght.Vel.ydot,BdyFrm.RearAxl.Rght.Vel.zdot
  Bus Selector3 : BusSelector  OutputSignals=InertFrm.FrntAxl.Lft.Vel.Xdot,InertFrm.FrntAxl.Lft.Vel.Ydot,InertFrm.FrntAxl.Lft.Vel.Zdot,InertFrm.FrntAxl.Rght.Vel.Xdot,InertFrm.FrntAxl.Rght.Vel.Ydot,InertFrm.FrntAxl.Rght.Vel.Zdot,InertFrm.RearAxl.Lft.Vel.Xdot,InertFrm.RearAxl.Lft.Vel.Ydot,InertFrm.RearAxl.Lft.Vel.Zdot,InertFrm.RearAxl.Rght.Vel.Xdot,InertFrm.RearAxl.Rght.Vel.Ydot,InertFrm.RearAxl.Rght.Vel.Zdot
  Inertial Frame CG to Axle Offset : Constant  Value=[zeros(2,4);VEH.HeightCG*ones(1,4)]
  Mux1 : Mux  Inputs=12
  Mux2 : Mux  Inputs=12
  Mux3 : Mux  Inputs=12
  Reshape : Reshape  OutputDimensionality=Customize  OutputDimensions=[3,4]
  Reshape1 : Reshape  OutputDimensionality=Customize  OutputDimensions=[3,4]
  Reshape2 : Reshape  OutputDimensionality=Customize  OutputDimensions=[3,4]
  Sum : Sum  Inputs=|+-
  VehSusp : Outport  VectorParamsAs1DForOutWhenUnconnected=off
  VehVbody : Outport  Port=2  VectorParamsAs1DForOutWhenUnconnected=off
  wires:
  Veh/1 -> Bus Selector3/1, Bus Selector2/1, Bus Selector1/1
  Reshape2/1 -> VehVbody/1  "V"
  Bus Creator3/1 -> VehSusp/1  "Veh"
  Reshape/1 -> Sum/1
  Bus Selector1/1 -> Mux2/1  "<X>"
  Bus Selector1/2 -> Mux2/2  "<Y>"
  Bus Selector1/3 -> Mux2/3  "<Z>"
  Bus Selector1/4 -> Mux2/4  "<X>"
  Bus Selector1/5 -> Mux2/5  "<Y>"
  Bus Selector1/6 -> Mux2/6  "<Z>"
  Bus Selector1/7 -> Mux2/7  "<X>"
  Bus Selector1/8 -> Mux2/8  "<Y>"
  Bus Selector1/9 -> Mux2/9  "<Z>"
  Bus Selector1/10 -> Mux2/10  "<X>"
  Bus Selector1/11 -> Mux2/11  "<Y>"
  Bus Selector1/12 -> Mux2/12  "<Z>"
  Bus Selector2/1 -> Mux1/1  "<xdot>"
  Bus Selector2/2 -> Mux1/2  "<ydot>"
  Bus Selector2/3 -> Mux1/3  "<zdot>"
  Bus Selector2/4 -> Mux1/4  "<xdot>"
  Bus Selector2/5 -> Mux1/5  "<ydot>"
  Bus Selector2/6 -> Mux1/6  "<zdot>"
  Bus Selector2/7 -> Mux1/7  "<xdot>"
  Bus Selector2/8 -> Mux1/8  "<ydot>"
  Bus Selector2/9 -> Mux1/9  "<zdot>"
  Bus Selector2/10 -> Mux1/10  "<xdot>"
  Bus Selector2/11 -> Mux1/11  "<ydot>"
  Bus Selector2/12 -> Mux1/12  "<zdot>"
  Mux1/1 -> Reshape2/1
  Mux2/1 -> Reshape/1
  Inertial Frame CG to Axle Offset/1 -> Sum/2
  Sum/1 -> Bus Creator3/1  "P"
  Mux3/1 -> Reshape1/1
  Bus Selector3/12 -> Mux3/12  "<Zdot>"
  Bus Selector3/11 -> Mux3/11  "<Ydot>"
  Bus Selector3/10 -> Mux3/10  "<Xdot>"
  Bus Selector3/9 -> Mux3/9  "<Zdot>"
  Bus Selector3/8 -> Mux3/8  "<Ydot>"
  Bus Selector3/7 -> Mux3/7  "<Xdot>"
  Bus Selector3/6 -> Mux3/6  "<Zdot>"
  Bus Selector3/5 -> Mux3/5  "<Ydot>"
  Bus Selector3/4 -> Mux3/4  "<Xdot>"
  Bus Selector3/3 -> Mux3/3  "<Zdot>"
  Bus Selector3/2 -> Mux3/2  "<Ydot>"
  Bus Selector3/1 -> Mux3/1  "<Xdot>"
  Reshape1/1 -> Bus Creator3/2  "V"

== system PassVeh14DOF/Suspension/MacPherson Suspension/Wheel  Adapter ==
  Wheels : Inport
  Bus Selector : BusSelector  OutputSignals=SuspFrame.Fx,SuspFrame.Fy
  Bus Selector1 : BusSelector  OutputSignals=SuspFrame.RL
  Bus Selector2 : BusSelector  OutputSignals=SuspFrame.Mx,SuspFrame.My,SuspFrame.Mz
  Bus Selector3 : BusSelector  OutputSignals=SuspFrame.z,SuspFrame.zdot
  Matrix Concatenate : Concatenate  NumInputs=3  Mode=Multidimensional array
  Reshape{,1..7} (8 alike) : Reshape  OutputDimensionality=Row vector (2-D)
  WhlFx : Outport  VectorParamsAs1DForOutWhenUnconnected=off
  WhlFy : Outport  Port=2  VectorParamsAs1DForOutWhenUnconnected=off
  z : Outport  Port=3  VectorParamsAs1DForOutWhenUnconnected=off
  zdot : Outport  Port=4  VectorParamsAs1DForOutWhenUnconnected=off
  M : Outport  Port=5  VectorParamsAs1DForOutWhenUnconnected=off
  RL : Outport  Port=6  VectorParamsAs1DForOutWhenUnconnected=off
  wires:
  Reshape7/1 -> WhlFy/1
  Reshape6/1 -> WhlFx/1
  Bus Selector/1 -> Reshape6/1  "<Fx>"
  Bus Selector/2 -> Reshape7/1  "<Fy>"
  Bus Selector3/1 -> Reshape/1  "<z>"
  Wheels/1 -> Bus Selector1/1, Bus Selector2/1, Bus Selector3/1, Bus Selector/1
  Bus Selector3/2 -> Reshape2/1  "<zdot>"
  Reshape2/1 -> zdot/1  "zdot"
  Bus Selector1/1 -> Reshape1/1  "<RL>"
  Reshape1/1 -> RL/1  "RL"
  Bus Selector2/1 -> Reshape3/1  "<Mx>"
  Bus Selector2/2 -> Reshape4/1  "<My>"
  Bus Selector2/3 -> Reshape5/1  "<Mz>"
  Reshape3/1 -> Matrix Concatenate/1
  Reshape4/1 -> Matrix Concatenate/2
  Reshape5/1 -> Matrix Concatenate/3
  Matrix Concatenate/1 -> M/1  "M"
  Reshape/1 -> z/1  "z"

== system PassVeh14DOF/Suspension/Mapped Suspension/Steer Rate Adapter ==
  Veh : Inport
  Add : Sum
  Bus Selector3 : BusSelector  OutputSignals=BdyFrm.Cg.AngVel.r
  Constant : Constant  Value=zeros(1,4)
  Matrix Concatenate : Concatenate  NumInputs=3  Mode=Multidimensional array
  Matrix Concatenate1 : Concatenate  NumInputs=3  Mode=Multidimensional array
  Reshape2 : Reshape  OutputDimensionality=Row vector (2-D)
  Reshape3 : Reshape  OutputDimensionality=Row vector (2-D)
  Reshape4 : Reshape  OutputDimensionality=Row vector (2-D)
  Selector3 : Selector  InputPortWidth=1  IndexOptions=Index vector (dialog)  Indices=[1 1 1 1]  OutputSizes=1
  SteerRates : Constant  Value=zeros(1,4)
  AngVel : Outport  VectorParamsAs1DForOutWhenUnconnected=off
  wires:
  Reshape2/1 -> Matrix Concatenate1/1, Matrix Concatenate1/3, Matrix Concatenate1/2
  Constant/1 -> Reshape3/1
  Selector3/1 -> Reshape4/1
  Bus Selector3/1 -> Selector3/1  "<r>"
  Matrix Concatenate/1 -> Add/2
  SteerRates/1 -> Reshape2/1
  Reshape4/1 -> Matrix Concatenate/3
  Reshape3/1 -> Matrix Concatenate/2, Matrix Concatenate/1
  Matrix Concatenate1/1 -> Add/1
  Veh/1 -> Bus Selector3/1
  Add/1 -> AngVel/1  "AngVel"

== system PassVeh14DOF/Suspension/Mapped Suspension/Vehicle Adapter ==
  Veh : Inport
  Bus Creator3 : BusCreator  Inputs=2
  Bus Selector1 : BusSelector  OutputSignals=InertFrm.FrntAxl.Lft.Disp.X,InertFrm.FrntAxl.Lft.Disp.Y,InertFrm.FrntAxl.Lft.Disp.Z,InertFrm.FrntAxl.Rght.Disp.X,InertFrm.FrntAxl.Rght.Disp.Y,InertFrm.FrntAxl.Rght.Disp.Z,InertFrm.RearAxl.Lft.Disp.X,InertFrm.RearAxl.Lft.Disp.Y,InertFrm.RearAxl.Lft.Disp.Z,InertFrm.RearAxl.Rght.Disp.X,InertFrm.RearAxl.Rght.Disp.Y,InertFrm.RearAxl.Rght.Disp.Z
  Bus Selector2 : BusSelector  OutputSignals=BdyFrm.FrntAxl.Lft.Vel.xdot,BdyFrm.FrntAxl.Lft.Vel.ydot,BdyFrm.FrntAxl.Lft.Vel.zdot,BdyFrm.FrntAxl.Rght.Vel.xdot,BdyFrm.FrntAxl.Rght.Vel.ydot,BdyFrm.FrntAxl.Rght.Vel.zdot,BdyFrm.RearAxl.Lft.Vel.xdot,BdyFrm.RearAxl.Lft.Vel.ydot,BdyFrm.RearAxl.Lft.Vel.zdot,BdyFrm.RearAxl.Rght.Vel.xdot,BdyFrm.RearAxl.Rght.Vel.ydot,BdyFrm.RearAxl.Rght.Vel.zdot
  Bus Selector3 : BusSelector  OutputSignals=InertFrm.FrntAxl.Lft.Vel.Xdot,InertFrm.FrntAxl.Lft.Vel.Ydot,InertFrm.FrntAxl.Lft.Vel.Zdot,InertFrm.FrntAxl.Rght.Vel.Xdot,InertFrm.FrntAxl.Rght.Vel.Ydot,InertFrm.FrntAxl.Rght.Vel.Zdot,InertFrm.RearAxl.Lft.Vel.Xdot,InertFrm.RearAxl.Lft.Vel.Ydot,InertFrm.RearAxl.Lft.Vel.Zdot,InertFrm.RearAxl.Rght.Vel.Xdot,InertFrm.RearAxl.Rght.Vel.Ydot,InertFrm.RearAxl.Rght.Vel.Zdot
  Inertial Frame CG to Axle Offset : Constant  Value=[zeros(2,4);VEH.HeightCG*ones(1,4)]
  Mux1 : Mux  Inputs=12
  Mux2 : Mux  Inputs=12
  Mux3 : Mux  Inputs=12
  Reshape : Reshape  OutputDimensionality=Customize  OutputDimensions=[3,4]
  Reshape1 : Reshape  OutputDimensionality=Customize  OutputDimensions=[3,4]
  Reshape2 : Reshape  OutputDimensionality=Customize  OutputDimensions=[3,4]
  Sum : Sum  Inputs=|+-
  VehSusp : Outport  VectorParamsAs1DForOutWhenUnconnected=off
  VehVbody : Outport  Port=2  VectorParamsAs1DForOutWhenUnconnected=off
  wires:
  Veh/1 -> Bus Selector3/1, Bus Selector2/1, Bus Selector1/1
  Reshape2/1 -> VehVbody/1  "V"
  Bus Creator3/1 -> VehSusp/1  "Veh"
  Reshape/1 -> Sum/1
  Bus Selector1/1 -> Mux2/1  "<X>"
  Bus Selector1/2 -> Mux2/2  "<Y>"
  Bus Selector1/3 -> Mux2/3  "<Z>"
  Bus Selector1/4 -> Mux2/4  "<X>"
  Bus Selector1/5 -> Mux2/5  "<Y>"
  Bus Selector1/6 -> Mux2/6  "<Z>"
  Bus Selector1/7 -> Mux2/7  "<X>"
  Bus Selector1/8 -> Mux2/8  "<Y>"
  Bus Selector1/9 -> Mux2/9  "<Z>"
  Bus Selector1/10 -> Mux2/10  "<X>"
  Bus Selector1/11 -> Mux2/11  "<Y>"
  Bus Selector1/12 -> Mux2/12  "<Z>"
  Bus Selector2/1 -> Mux1/1  "<xdot>"
  Bus Selector2/2 -> Mux1/2  "<ydot>"
  Bus Selector2/3 -> Mux1/3  "<zdot>"
  Bus Selector2/4 -> Mux1/4  "<xdot>"
  Bus Selector2/5 -> Mux1/5  "<ydot>"
  Bus Selector2/6 -> Mux1/6  "<zdot>"
  Bus Selector2/7 -> Mux1/7  "<xdot>"
  Bus Selector2/8 -> Mux1/8  "<ydot>"
  Bus Selector2/9 -> Mux1/9  "<zdot>"
  Bus Selector2/10 -> Mux1/10  "<xdot>"
  Bus Selector2/11 -> Mux1/11  "<ydot>"
  Bus Selector2/12 -> Mux1/12  "<zdot>"
  Mux1/1 -> Reshape2/1
  Mux2/1 -> Reshape/1
  Inertial Frame CG to Axle Offset/1 -> Sum/2
  Sum/1 -> Bus Creator3/1  "P"
  Mux3/1 -> Reshape1/1
  Bus Selector3/12 -> Mux3/12  "<Zdot>"
  Bus Selector3/11 -> Mux3/11  "<Ydot>"
  Bus Selector3/10 -> Mux3/10  "<Xdot>"
  Bus Selector3/9 -> Mux3/9  "<Zdot>"
  Bus Selector3/8 -> Mux3/8  "<Ydot>"
  Bus Selector3/7 -> Mux3/7  "<Xdot>"
  Bus Selector3/6 -> Mux3/6  "<Zdot>"
  Bus Selector3/5 -> Mux3/5  "<Ydot>"
  Bus Selector3/4 -> Mux3/4  "<Xdot>"
  Bus Selector3/3 -> Mux3/3  "<Zdot>"
  Bus Selector3/2 -> Mux3/2  "<Ydot>"
  Bus Selector3/1 -> Mux3/1  "<Xdot>"
  Reshape1/1 -> Bus Creator3/2  "V"

== system PassVeh14DOF/Suspension/Mapped Suspension/Wheel  Adapter ==
  Wheels : Inport
  Bus Selector : BusSelector  OutputSignals=SuspFrame.Fx,SuspFrame.Fy
  Bus Selector1 : BusSelector  OutputSignals=SuspFrame.RL
  Bus Selector2 : BusSelector  OutputSignals=SuspFrame.Mx,SuspFrame.My,SuspFrame.Mz
  Bus Selector3 : BusSelector  OutputSignals=SuspFrame.z,SuspFrame.zdot
  Matrix Concatenate : Concatenate  NumInputs=3  Mode=Multidimensional array
  Reshape{,1..7} (8 alike) : Reshape  OutputDimensionality=Row vector (2-D)
  WhlFx : Outport  VectorParamsAs1DForOutWhenUnconnected=off
  WhlFy : Outport  Port=2  VectorParamsAs1DForOutWhenUnconnected=off
  z : Outport  Port=3  VectorParamsAs1DForOutWhenUnconnected=off
  zdot : Outport  Port=4  VectorParamsAs1DForOutWhenUnconnected=off
  M : Outport  Port=5  VectorParamsAs1DForOutWhenUnconnected=off
  RL : Outport  Port=6  VectorParamsAs1DForOutWhenUnconnected=off
  wires:
  Reshape7/1 -> WhlFy/1
  Reshape6/1 -> WhlFx/1
  Bus Selector/1 -> Reshape6/1  "<Fx>"
  Bus Selector/2 -> Reshape7/1  "<Fy>"
  Bus Selector3/1 -> Reshape/1  "<z>"
  Wheels/1 -> Bus Selector1/1, Bus Selector2/1, Bus Selector3/1, Bus Selector/1
  Bus Selector3/2 -> Reshape2/1  "<zdot>"
  Reshape2/1 -> zdot/1  "zdot"
  Bus Selector1/1 -> Reshape1/1  "<RL>"
  Reshape1/1 -> RL/1  "RL"
  Bus Selector2/1 -> Reshape3/1  "<Mx>"
  Bus Selector2/2 -> Reshape4/1  "<My>"
  Bus Selector2/3 -> Reshape5/1  "<Mz>"
  Reshape3/1 -> Matrix Concatenate/1
  Reshape4/1 -> Matrix Concatenate/2
  Reshape5/1 -> Matrix Concatenate/3
  Matrix Concatenate/1 -> M/1  "M"
  Reshape/1 -> z/1  "z"
